simulink model "nmpc_controller"  (R2026a)
settings: Solver=FixedStepAuto  StopTime=Inf  FixedStep=0.05
PostLoadFcn:
  | if any(exist('dsrtsu_mdlpostloadfcn', 'file') ~= 0), dsrtsu_mdlpostloadfcn('Execute', bdroot); end
InitFcn:
  | , if any(exist('rtifpga_mdlclblib', 'file') ~= 0), rtifpga_mdlclblib('Init', bdroot); end,
  | , if any(exist('dsmpb_private', 'file') ~= 0), dsmpb_private('dsmpb_mdlclblib', 'Init', bdroot); end,
model workspace (MAT data in the model file):
  controllerConfig.schema_version = 1
  controllerConfig.vehicle.m = 1723
  controllerConfig.vehicle.Iz = 1960
  controllerConfig.vehicle.lf = 1.232
  controllerConfig.vehicle.lr = 1.468
  controllerConfig.vehicle.Cy = 62700
  controllerConfig.vehicle.track = 1.539
  controllerConfig.vehicle.Rw = 0.31
  controllerConfig.vehicle.g = 9.81
  controllerConfig.Ts = 0.05
  controllerConfig.N = 40
  controllerConfig.nx = 5
  controllerConfig.nu = 3
  controllerConfig.np = 19
  controllerConfig.W = [20  0  0  0  0  0  0  0; 0  50  0  0  0  0  0  0; 0  0  2  0  0  0  0  0; 0  0  0  0.1  0  0  0  0; 0  0  0  0  0.1  0  0  0; 0  0  0  0  0  1e-06  0  0; 0  0  0  0  0  0  1e-06  0; 0  0  0  0  0  0  0  1e-07]
  controllerConfig.We = [200  0  0  0  0; 0  500  0  0  0; 0  0  20  0  0; 0  0  0  1  0; 0  0  0  0  1]
  controllerConfig.lbu = [-9000; -9000; -6000]
  controllerConfig.ubu = [4500; 9000; 6000]
  controllerConfig.slack_linear = 1000
  controllerConfig.slack_quadratic = 1000
  controllerConfig.max_iter = 200
  controllerConfig.tolerance = 1e-06
  controllerConfig.qp_max_iter = 100
  controllerConfig.cond_N = 10
  initialUguess = [0  0  0  0  0  0  0  0  0  0  0  0  0  0  0  0  0  0  0  0  0  0  0  0  0  0  0  0  0  0  0  0  0  0  0  0  0  0  0  0; 0  0  0  0  0  0  0  0  0  0  0  0  0  0  0  0  0  0  0  0  0  0  0  0  0  0  0  0  0  0  0  0  0  0  0  0  0  0  0  0; 0  0  0  0  0  0  0  0  0  0  0  0  0  0  0  0  0  0  0  0  0  0  0  0  0  0  0  0  0  0  0  0  0  0  0  0  0  0  0  0]
  initialXguess = [-0.116260692271  -0.116260692271  -0.116260692271  -0.116260692271  -0.116260692271  -0.116260692271  -0.116260692271  -0.116260692271  -0.116260692271  -0.116260692271  -0.116260692271  -0.116260692271  -0.116260692271  -0.116260692271  -0.116260692271  -0.116260692271  -0.116260692271  -0.116260692271  -0.116260692271  -0.116260692271  -0.116260692271  -0.116260692271  -0.116260692271  -0.116260692271  -0.116260692271  -0.116260692271  -0.116260692271  -0.116260692271  -0.116260692271  -0.116260692271  -0.116260692271  -0.116260692271  -0.116260692271  -0.116260692271  -0.116260692271  -0.116260692271  -0.116260692271  -0.116260692271  -0.116260692271  -0.116260692271  -0.116260692271; -0.0164016572522  -0.0164016572522  -0.0164016572522  -0.0164016572522  -0.0164016572522  -0.0164016572522  -0.0164016572522  -0.0164016572522  -0.0164016572522  -0.0164016572522  -0.0164016572522  -0.0164016572522  -0.0164016572522  -0.0164016572522  -0.0164016572522  -0.0164016572522  -0.0164016572522  -0.0164016572522  -0.0164016572522  -0.0164016572522  -0.0164016572522  -0.0164016572522  -0.0164016572522  -0.0164016572522  -0.0164016572522  -0.0164016572522  -0.0164016572522  -0.0164016572522  -0.0164016572522  -0.0164016572522  -0.0164016572522  -0.0164016572522  -0.0164016572522  -0.0164016572522  -0.0164016572522  -0.0164016572522  -0.0164016572522  -0.0164016572522  -0.0164016572522  -0.0164016572522  -0.0164016572522; 0  0  0  0  0  0  0  0  0  0  0  0  0  0  0  0  0  0  0  0  0  0  0  0  0  0  0  0  0  0  0  0  0  0  0  0  0  0  0  0  0; 0  0  0  0  0  0  0  0  0  0  0  0  0  0  0  0  0  0  0  0  0  0  0  0  0  0  0  0  0  0  0  0  0  0  0  0  0  0  0  0  0; 0  0  0  0  0  0  0  0  0  0  0  0  0  0  0  0  0  0  0  0  0  0  0  0  0  0  0  0  0  0  0  0  0  0  0  0  0  0  0  0  0]
  instance.schema_version = 1
  instance.family_id = 1
  instance.instance_id = 1
  instance.seed = 1001
  instance.draws.uniform_draws = [0.306232179549 0.265063565608 0.196060063151 0.430521476567 0.0231135519921 0.195781915084 0.352805288469]
  instance.draws.e0_m = -0.116260692271
  instance.draws.psi0_rad = -0.0164016572522
  instance.draws.vx0_mps = 21.9606006315
  instance.draws.d0_m = 33.6104295313
  instance.draws.alead_mps2 = -5.93065934402
  instance.draws.vt_mps = 13.3310740371
  instance.draws.dt_m = 23.8201322117
  instance.draws.kc_per_m = 0
  instance.draws.curvature_choice_index = []
  instance.road.lane_width_m = 3.75
  instance.road.curvature_per_m = 0
  instance.road.bounds_m = [-1.75; 5.25]
  instance.friction_coefficient = 0.9
  instance.reference.speed_mps = 21.9606006315
  instance.timing.duration_s = 8
  instance.timing.controller_period_s = 0.05
  instance.timing.plant_step_s = 0.001
  instance.timing.number_of_control_samples = 160
  instance.ego.initial_state = [-0.116260692271; -0.0164016572522; 0; 0; 0]
  instance.ego.initial_longitudinal_speed_mps = 21.9606006315
  instance.ego.initial_station_m = 0
  instance.obstacles(1).initial_station_m = 33.6104295313
  instance.obstacles(1).lateral_position_m = 0
  instance.obstacles(1).initial_speed_mps = 21.9606006315
  instance.obstacles(1).acceleration_mps2 = -5.93065934402
  instance.obstacles(1).braking_start_s = 1
  instance.obstacles(2).initial_station_m = 23.8201322117
  instance.obstacles(2).lateral_position_m = 3.75
  instance.obstacles(2).initial_speed_mps = 13.3310740371
  instance.obstacles(2).acceleration_mps2 = 0
  instance.obstacles(2).braking_start_s = 0
  instance.obstacle_geometry.safety_semi_axes_m = [1.3; 4.5]
  instance.obstacle_geometry.collision_semi_axes_m = [0.9; 2.5]
  instance.termination.run_off_limit_m = 6
  laneData.schema_version = 1
  laneData.instance.schema_version = 1
  laneData.instance.family_id = 1
  laneData.instance.instance_id = 1
  laneData.instance.seed = 1001
  laneData.instance.draws.uniform_draws = [0.306232179549 0.265063565608 0.196060063151 0.430521476567 0.0231135519921 0.195781915084 0.352805288469]
  laneData.instance.draws.e0_m = -0.116260692271
  laneData.instance.draws.psi0_rad = -0.0164016572522
  laneData.instance.draws.vx0_mps = 21.9606006315
  laneData.instance.draws.d0_m = 33.6104295313
  laneData.instance.draws.alead_mps2 = -5.93065934402
  laneData.instance.draws.vt_mps = 13.3310740371
  laneData.instance.draws.dt_m = 23.8201322117
  laneData.instance.draws.kc_per_m = 0
  laneData.instance.draws.curvature_choice_index = []
  laneData.instance.road.lane_width_m = 3.75
  laneData.instance.road.curvature_per_m = 0
  laneData.instance.road.bounds_m = [-1.75; 5.25]
  laneData.instance.friction_coefficient = 0.9
  laneData.instance.reference.speed_mps = 21.9606006315
  laneData.instance.timing.duration_s = 8
  laneData.instance.timing.controller_period_s = 0.05
  laneData.instance.timing.plant_step_s = 0.001
  laneData.instance.timing.number_of_control_samples = 160
  laneData.instance.ego.initial_state = [-0.116260692271; -0.0164016572522; 0; 0; 0]
  laneData.instance.ego.initial_longitudinal_speed_mps = 21.9606006315
  laneData.instance.ego.initial_station_m = 0
  laneData.instance.obstacles(1).initial_station_m = 33.6104295313
  laneData.instance.obstacles(1).lateral_position_m = 0
  laneData.instance.obstacles(1).initial_speed_mps = 21.9606006315
  laneData.instance.obstacles(1).acceleration_mps2 = -5.93065934402
  laneData.instance.obstacles(1).braking_start_s = 1
  laneData.instance.obstacles(2).initial_station_m = 23.8201322117
  laneData.instance.obstacles(2).lateral_position_m = 3.75
  laneData.instance.obstacles(2).initial_speed_mps = 13.3310740371
  laneData.instance.obstacles(2).acceleration_mps2 = 0
  laneData.instance.obstacles(2).braking_start_s = 0
  laneData.instance.obstacle_geometry.safety_semi_axes_m = [1.3; 4.5]
  laneData.instance.obstacle_geometry.collision_semi_axes_m = [0.9; 2.5]
  laneData.instance.termination.run_off_limit_m = 6
  laneData.vehicle.m = 1723
  laneData.vehicle.Iz = 1960
  laneData.vehicle.lf = 1.232
  laneData.vehicle.lr = 1.468
  laneData.vehicle.Cy = 62700
  laneData.vehicle.track = 1.539
  laneData.vehicle.Rw = 0.31
  laneData.vehicle.g = 9.81
  laneData.lanes.schema_version = 1
  laneData.lanes.family_id = 1
  laneData.lanes.instance_id = 1
  laneData.lanes.station_m = [0 0.01 0.02 0.03 0.04 0.05 0.06 0.07 0.08 0.09 0.1 0.11 ... (50001 elements, 50001x1)]
  laneData.lanes.lane_width_m = 3.75
  laneData.lanes.number_of_lanes = 2
  laneData.lanes.curvature_per_m = 0
  laneData.lanes.origin_pose = [0; 0; 0]
  laneData.lanes.reference.X_m = [0 0.01 0.02 0.03 0.04 0.05 0.06 0.07 0.08 0.09 0.1 0.11 ... (50001 elements, 50001x1)]
  laneData.lanes.reference.Y_m = [0 0 0 0 0 0 0 0 0 0 0 0 ... (50001 elements, 50001x1)]
  laneData.lanes.reference.heading_rad = [0 0 0 0 0 0 0 0 0 0 0 0 ... (50001 elements, 50001x1)]
  laneData.lanes.boundaries.offsets_m = [-1.875; 1.875; 5.625]
  laneData.lanes.boundaries.X_m = [0 0.01 0.02 0.03 0.04 0.05 0.06 0.07 0.08 0.09 0.1 0.11 ... (150003 elements, 50001x3)]
  laneData.lanes.boundaries.Y_m = [-1.875 -1.875 -1.875 -1.875 -1.875 -1.875 -1.875 -1.875 -1.875 -1.875 -1.875 -1.875 ... (150003 elements, 50001x3)]
  laneData.lanes.centerlines.offsets_m = [0; 3.75]
  laneData.lanes.centerlines.X_m = [0 0.01 0.02 0.03 0.04 0.05 0.06 0.07 0.08 0.09 0.1 0.11 ... (100002 elements, 50001x2)]
  laneData.lanes.centerlines.Y_m = [0 0 0 0 0 0 0 0 0 0 0 0 ... (100002 elements, 50001x2)]
  laneData.lanes.controller_bounds.offsets_m = [-1.75; 5.25]
  laneData.lanes.controller_bounds.X_m = [0 0.01 0.02 0.03 0.04 0.05 0.06 0.07 0.08 0.09 0.1 0.11 ... (100002 elements, 50001x2)]
  laneData.lanes.controller_bounds.Y_m = [-1.75 -1.75 -1.75 -1.75 -1.75 -1.75 -1.75 -1.75 -1.75 -1.75 -1.75 -1.75 ... (100002 elements, 50001x2)]
  laneData.reference.station_m = [0 0.01 0.02 0.03 0.04 0.05 0.06 0.07 0.08 0.09 0.1 0.11 ... (50001 elements, 50001x1)]
  laneData.reference.X_m = [0 0.01 0.02 0.03 0.04 0.05 0.06 0.07 0.08 0.09 0.1 0.11 ... (50001 elements, 50001x1)]
  laneData.reference.Y_m = [0 0 0 0 0 0 0 0 0 0 0 0 ... (50001 elements, 50001x1)]
  laneData.reference.heading_rad = [0 0 0 0 0 0 0 0 0 0 0 0 ... (50001 elements, 50001x1)]
  laneData.reference.curvature_per_m = [0 0 0 0 0 0 0 0 0 0 0 0 ... (50001 elements, 50001x1)]
  laneData.reference.psi_pvr = [0 0 0 0 0 0 0 0 0 0 0 0 ... (50001 elements, 50001x1)]
  laneData.reference.dpsi_pr = [0 0 0 0 0 0 0 0 0 0 0 0 ... (50001 elements, 50001x1)]
  laneData.reference.dpsi_pvr = [0 0 0 0 0 0 0 0 0 0 0 0 ... (50001 elements, 50001x1)]
  laneData.reference.ddpsi_pr = [0 0 0 0 0 0 0 0 0 0 0 0 ... (50001 elements, 50001x1)]
  laneData.reference.ddpsi_pvr = [0 0 0 0 0 0 0 0 0 0 0 0 ... (50001 elements, 50001x1)]
  laneData.reference.vr = [21.9606006315 21.9606006315 21.9606006315 21.9606006315 21.9606006315 21.9606006315 21.9606006315 21.9606006315 21.9606006315 21.9606006315 21.9606006315 21.9606006315 ... (50001 elements, 50001x1)]
  laneData.reference.dvr = [0 0 0 0 0 0 0 0 0 0 0 0 ... (50001 elements, 50001x1)]
  laneData.reference.emin = [-1.75 -1.75 -1.75 -1.75 -1.75 -1.75 -1.75 -1.75 -1.75 -1.75 -1.75 -1.75 ... (50001 elements, 50001x1)]
  laneData.reference.emax = [5.25 5.25 5.25 5.25 5.25 5.25 5.25 5.25 5.25 5.25 5.25 5.25 ... (50001 elements, 50001x1)]
  mu = 0.9
PreSaveFcn:
  | , if any(exist('dsmpb_private', 'file') ~= 0), dsmpb_private('dsmpb_mdlclblib', 'PreSave', bdroot); end,
CloseFcn:
  | , if any(exist('dsmpb_private', 'file') ~= 0), dsmpb_private('dsmpb_mdlclblib', 'Close', bdroot); end,
settings Model: DataDictionary=vehicle_control.sldd  DSRTSU_INTERNAL_RTIFPGA=231  DSRTSU_INTERNAL_RTISTBM_VER=26.1  Creator=rayyu  LastModifiedBy=bxr240009
settings OptimizationCC: ConditionallyExecuteInputs=off  OptimizeBlockIOStorage=off  BufferReuse=off  InitFltsAndDblsToZero=on
settings DebuggingCC: TasksWithSamePriorityMsg=none
settings HardwareCC: ProdLargestAtomicInteger=Integer  ProdHWDeviceType=Custom Processor->Custom
settings ModelReferenceCC: EnableParallelModelReferenceBuilds=on
settings RTWCC: SystemTargetFile=dsrt.tlc  GenCodeOnly=on  TemplateMakefile=dsrt_default_tmf  RTWVerbose=off  Description=dSPACE Target DSRT - Generates SIC files for import by ConfigurationDesk and VEOS. Provides code generation for Simulink models imported in ConfigurationDesk.
settings RTWCC: CustomInclude=|
  | "C:\Users\bxr240009\Downloads\bim\real-time-performance-analysis\dependencies\acados-veos\include"
  | "C:\Users\bxr240009\Downloads\bim\real-time-performance-analysis\dependencies\acados-veos\include\blasfeo\include"
  | "C:\Users\bxr240009\Downloads\bim\real-time-performance-analysis\dependencies\acados-veos\include\hpipm\include"
settings RTWCC: CustomSource=|
  | C:\Users\bxr240009\Downloads\bim\real-time-performance-analysis\build\desktop\controller\c_generated_code\acados_sim_solver_ecu_vehicle_nmpc.c
  | C:\Users\bxr240009\Downloads\bim\real-time-performance-analysis\build\desktop\controller\c_generated_code\acados_solver_ecu_vehicle_nmpc.c
  | C:\Users\bxr240009\Downloads\bim\real-time-performance-analysis\build\desktop\controller\c_generated_code\ecu_vehicle_nmpc_constraints\ecu_vehicle_nmpc_constr_h_0_fun.c
  | C:\Users\bxr240009\Downloads\bim\real-time-performance-analysis\build\desktop\controller\c_generated_code\ecu_vehicle_nmpc_constraints\ecu_vehicle_nmpc_constr_h_0_fun_jac_uxt_zt.c
  | C:\Users\bxr240009\Downloads\bim\real-time-performance-analysis\build\desktop\controller\c_generated_code\ecu_vehicle_nmpc_constraints\ecu_vehicle_nmpc_constr_h_fun.c
  | C:\Users\bxr240009\Downloads\bim\real-time-performance-analysis\build\desktop\controller\c_generated_code\ecu_vehicle_nmpc_constraints\ecu_vehicle_nmpc_constr_h_fun_jac_uxt_zt.c
  | C:\Users\bxr240009\Downloads\bim\real-time-performance-analysis\build\desktop\controller\c_generated_code\ecu_vehicle_nmpc_cost\ecu_vehicle_nmpc_cost_y_0_fun.c
  | C:\Users\bxr240009\Downloads\bim\real-time-performance-analysis\build\desktop\controller\c_generated_code\ecu_vehicle_nmpc_cost\ecu_vehicle_nmpc_cost_y_0_fun_jac_ut_xt.c
  | C:\Users\bxr240009\Downloads\bim\real-time-performance-analysis\build\desktop\controller\c_generated_code\ecu_vehicle_nmpc_cost\ecu_vehicle_nmpc_cost_y_e_fun.c
  | C:\Users\bxr240009\Downloads\bim\real-time-performance-analysis\build\desktop\controller\c_generated_code\ecu_vehicle_nmpc_cost\ecu_vehicle_nmpc_cost_y_e_fun_jac_ut_xt.c
  | C:\Users\bxr240009\Downloads\bim\real-time-performance-analysis\build\desktop\controller\c_generated_code\ecu_vehicle_nmpc_cost\ecu_vehicle_nmpc_cost_y_fun.c
  | C:\Users\bxr240009\Downloads\bim\real-time-performance-analysis\build\desktop\controller\c_generated_code\ecu_vehicle_nmpc_cost\ecu_vehicle_nmpc_cost_y_fun_jac_ut_xt.c
  | C:\Users\bxr240009\Downloads\bim\real-time-performance-analysis\build\desktop\controller\c_generated_code\ecu_vehicle_nmpc_model\ecu_vehicle_nmpc_expl_ode_fun.c
  | C:\Users\bxr240009\Downloads\bim\real-time-performance-analysis\build\desktop\controller\c_generated_code\ecu_vehicle_nmpc_model\ecu_vehicle_nmpc_expl_vde_adj.c
  | C:\Users\bxr240009\Downloads\bim\real-time-performance-analysis\build\desktop\controller\c_generated_code\ecu_vehicle_nmpc_model\ecu_vehicle_nmpc_expl_vde_forw.c
settings RTWCC: CustomLibrary=|
  | "C:\Users\bxr240009\Downloads\bim\real-time-performance-analysis\dependencies\acados-veos\lib\acados.lib"
  | "C:\Users\bxr240009\Downloads\bim\real-time-performance-analysis\dependencies\acados-veos\lib\blasfeo.lib"
  | "C:\Users\bxr240009\Downloads\bim\real-time-performance-analysis\dependencies\acados-veos\lib\hpipm.lib"
settings STFCustomTargetCC: SystemTargetFile=dsrt.tlc  MultiwordLength=2048.0  ParMdlRefBuildCompliant=on  GRTInterface=off  DSTargetArchitecture=32-bit  TRCGenerateVirtualBlocks=off  TRCGenerateLabels=off  TRCOnlyGlobals=off  VDFType=TRC  TRCGenerateParamValues=off  TRCGenerateDerivatives=off  TRCGenerateStates=off  TRCIsOmitVdOn=on
settings GRTTargetCC: CompOptLevelCompliant=off  ConcurrentExecutionCompliant=off  CombineOutputUpdateFcns=off  MatFileLogging=off  CPPClassGenCompliant=off

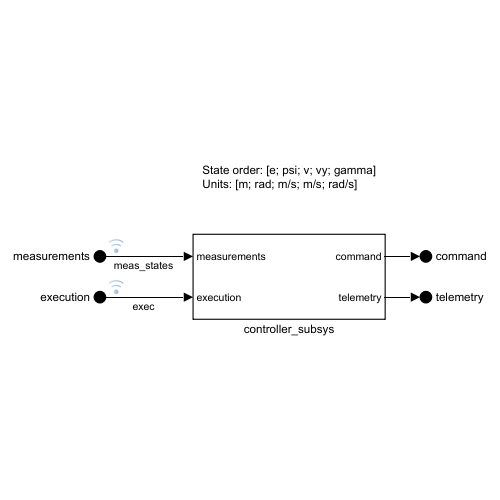
[thumbnail: Simulink's stored preview of the top-level diagram]
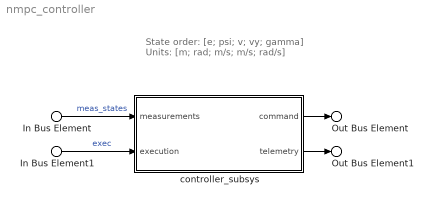
== system nmpc_controller ==
  note: State order: [e; psi; v; vy; gamma]
      | Units: [m; rad; m/s; m/s; rad/s]
  In Bus Element : Inport  PortName=measurements
  In Bus Element1 : Inport  Port=2  PortName=execution
  controller_subsys : Subsystem
  Out Bus Element : Outport  PortName=command
  Out Bus Element1 : Outport  Port=2  PortName=telemetry
  wires:
  In Bus Element/1 -> controller_subsys/1(measurements)  "meas_states"
  In Bus Element1/1 -> controller_subsys/2(execution)  "exec"
  controller_subsys/1(command) -> Out Bus Element/1
  controller_subsys/2(telemetry) -> Out Bus Element1/1

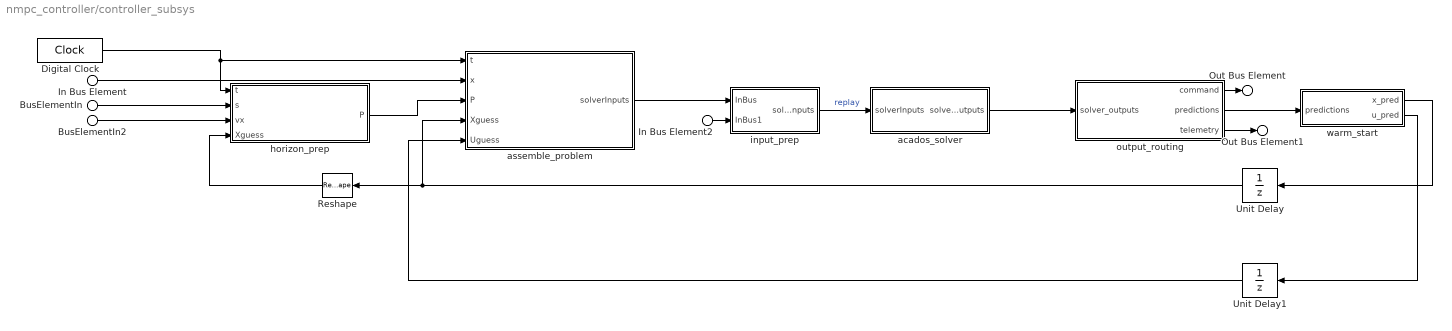
== system nmpc_controller/controller_subsys ==
  In Bus Element : Inport  PortName=measurements  Element=x
  BusElementIn2 : Inport  PortName=measurements  Element=vx
  BusElementIn : Inport  PortName=measurements  Element=s
  In Bus Element2 : Inport  Port=2  PortName=execution
  Digital Clock : DigitalClock  SampleTime=0.05
  Reshape : Reshape  OutputDimensionality=Customize  OutputDimensions=[205,1]
  Unit Delay : UnitDelay  SampleTime=0.05
  Unit Delay1 : UnitDelay  SampleTime=0.05
  acados_solver : Subsystem
  assemble_problem : MATLAB Function  TreatAsAtomicUnit=on
  horizon_prep : MATLAB Function  TreatAsAtomicUnit=on
  input_prep : Subsystem
  output_routing : Subsystem
  warm_start : Subsystem
  Out Bus Element : Outport  PortName=command
  Out Bus Element1 : Outport  Port=2  PortName=telemetry
  wires:
  acados_solver/1(solver_outputs) -> output_routing/1(solver_outputs)
  In Bus Element/1 -> assemble_problem/2(x)
  assemble_problem/1(solverInputs) -> input_prep/1(InBus)
  output_routing/2(predictions) -> warm_start/1(predictions)
  warm_start/1(x_pred) -> Unit Delay/1
  warm_start/2(u_pred) -> Unit Delay1/1
  input_prep/1(solverInputs) -> acados_solver/1(solverInputs)  "replay"
  horizon_prep/1(P) -> assemble_problem/3(P)
  BusElementIn2/1 -> horizon_prep/3(vx)
  BusElementIn/1 -> horizon_prep/2(s)
  output_routing/1(command) -> Out Bus Element/1
  output_routing/3(telemetry) -> Out Bus Element1/1
  In Bus Element2/1 -> input_prep/2(InBus1)
  Digital Clock/1 -> horizon_prep/1(t), assemble_problem/1(t)
  Unit Delay/1 -> assemble_problem/4(Xguess), Reshape/1
  Unit Delay1/1 -> assemble_problem/5(Uguess)
  Reshape/1 -> horizon_prep/4(Xguess)

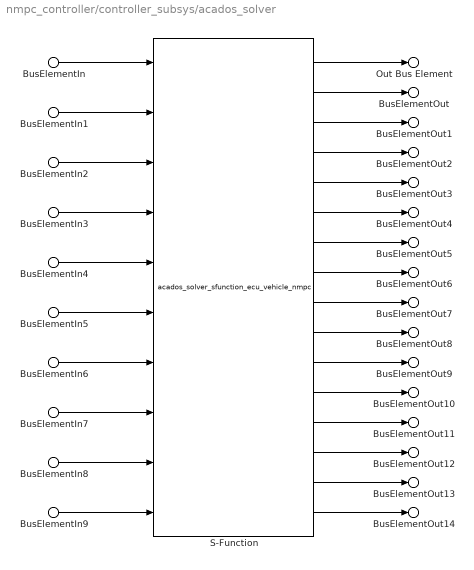
== system nmpc_controller/controller_subsys/acados_solver ==
  BusElementIn : Inport  PortName=solverInputs  Element=lbx_0
  BusElementIn1 : Inport  PortName=solverInputs  Element=ubx_0
  BusElementIn2 : Inport  PortName=solverInputs  Element=parameter_traj
  BusElementIn3 : Inport  PortName=solverInputs  Element=lh
  BusElementIn4 : Inport  PortName=solverInputs  Element=uh
  BusElementIn5 : Inport  PortName=solverInputs  Element=lh_0
  BusElementIn6 : Inport  PortName=solverInputs  Element=uh_0
  BusElementIn7 : Inport  PortName=solverInputs  Element=x_init
  BusElementIn8 : Inport  PortName=solverInputs  Element=u_init
  BusElementIn9 : Inport  PortName=solverInputs  Element=iter_cap
  S-Function : S-Function  FunctionName=acados_solver_sfunction_ecu_vehicle_nmpc  SFunctionDeploymentMode=off  EnableBusSupport=off
  Out Bus Element : Outport  PortName=solver_outputs  Element=u0
  BusElementOut : Outport  PortName=solver_outputs  Element=utraj
  BusElementOut1 : Outport  PortName=solver_outputs  Element=xtraj
  BusElementOut2 : Outport  PortName=solver_outputs  Element=slack_values
  BusElementOut3 : Outport  PortName=solver_outputs  Element=solver_status
  BusElementOut4 : Outport  PortName=solver_outputs  Element=cost_value
  BusElementOut5 : Outport  PortName=solver_outputs  Element=kkt_residuals
  BusElementOut6 : Outport  PortName=solver_outputs  Element=x1
  BusElementOut7 : Outport  PortName=solver_outputs  Element=cpu_time
  BusElementOut8 : Outport  PortName=solver_outputs  Element=cpu_time_qp
  BusElementOut9 : Outport  PortName=solver_outputs  Element=cpu_time_lin
  BusElementOut10 : Outport  PortName=solver_outputs  Element=sqp_iter
  BusElementOut11 : Outport  PortName=solver_outputs  Element=qp_iteration_history
  BusElementOut12 : Outport  PortName=solver_outputs  Element=residual_history
  BusElementOut13 : Outport  PortName=solver_outputs  Element=history_length
  BusElementOut14 : Outport  PortName=solver_outputs  Element=lam_stage0
  wires:
  BusElementIn4/1 -> S-Function/5
  BusElementIn2/1 -> S-Function/3
  BusElementIn8/1 -> S-Function/9
  BusElementIn6/1 -> S-Function/7
  BusElementIn5/1 -> S-Function/6
  BusElementIn7/1 -> S-Function/8
  BusElementIn1/1 -> S-Function/2
  BusElementIn/1 -> S-Function/1
  BusElementIn3/1 -> S-Function/4
  BusElementIn9/1 -> S-Function/10
  S-Function/9 -> BusElementOut7/1
  S-Function/1 -> Out Bus Element/1
  S-Function/15 -> BusElementOut13/1
  S-Function/14 -> BusElementOut12/1
  S-Function/3 -> BusElementOut1/1
  S-Function/4 -> BusElementOut2/1
  S-Function/8 -> BusElementOut6/1
  S-Function/2 -> BusElementOut/1
  S-Function/7 -> BusElementOut5/1
  S-Function/16 -> BusElementOut14/1
  S-Function/10 -> BusElementOut8/1
  S-Function/13 -> BusElementOut11/1
  S-Function/6 -> BusElementOut4/1
  S-Function/12 -> BusElementOut10/1
  S-Function/11 -> BusElementOut9/1
  S-Function/5 -> BusElementOut3/1

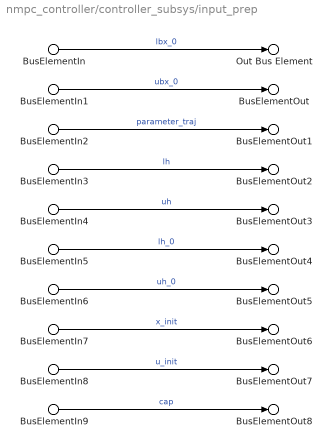
== system nmpc_controller/controller_subsys/input_prep ==
  BusElementIn : Inport  PortName=InBus  Element=lbx_0
  BusElementIn1 : Inport  PortName=InBus  Element=ubx_0
  BusElementIn2 : Inport  PortName=InBus  Element=parameter_traj
  BusElementIn3 : Inport  PortName=InBus  Element=lh
  BusElementIn4 : Inport  PortName=InBus  Element=uh
  BusElementIn5 : Inport  PortName=InBus  Element=lh_0
  BusElementIn6 : Inport  PortName=InBus  Element=uh_0
  BusElementIn7 : Inport  PortName=InBus  Element=x_init
  BusElementIn8 : Inport  PortName=InBus  Element=u_init
  BusElementIn9 : Inport  Port=2  PortName=InBus1  Element=cap
  Out Bus Element : Outport  PortName=solverInputs  Element=lbx_0
  BusElementOut : Outport  PortName=solverInputs  Element=ubx_0
  BusElementOut1 : Outport  PortName=solverInputs  Element=parameter_traj
  BusElementOut2 : Outport  PortName=solverInputs  Element=lh
  BusElementOut3 : Outport  PortName=solverInputs  Element=uh
  BusElementOut4 : Outport  PortName=solverInputs  Element=lh_0
  BusElementOut5 : Outport  PortName=solverInputs  Element=uh_0
  BusElementOut6 : Outport  PortName=solverInputs  Element=x_init
  BusElementOut7 : Outport  PortName=solverInputs  Element=u_init
  BusElementOut8 : Outport  PortName=solverInputs  Element=iter_cap
  wires:
  BusElementIn/1 -> Out Bus Element/1  "lbx_0"
  BusElementIn1/1 -> BusElementOut/1  "ubx_0"
  BusElementIn2/1 -> BusElementOut1/1  "parameter_traj"
  BusElementIn3/1 -> BusElementOut2/1  "lh"
  BusElementIn4/1 -> BusElementOut3/1  "uh"
  BusElementIn5/1 -> BusElementOut4/1  "lh_0"
  BusElementIn6/1 -> BusElementOut5/1  "uh_0"
  BusElementIn7/1 -> BusElementOut6/1  "x_init"
  BusElementIn8/1 -> BusElementOut7/1  "u_init"
  BusElementIn9/1 -> BusElementOut8/1  "cap"

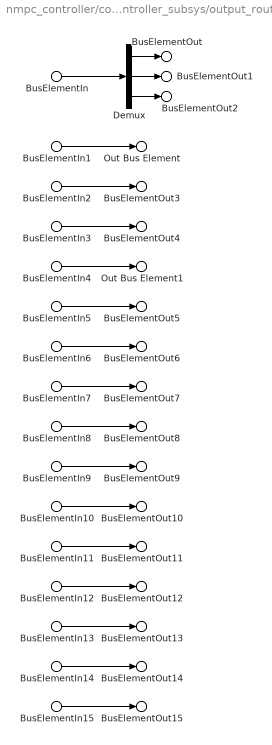
== system nmpc_controller/controller_subsys/output_routing ==
  BusElementIn : Inport  PortName=solver_outputs  Element=u0
  BusElementIn1 : Inport  PortName=solver_outputs  Element=utraj
  BusElementIn2 : Inport  PortName=solver_outputs  Element=xtraj
  BusElementIn4 : Inport  PortName=solver_outputs  Element=slack_values
  BusElementIn5 : Inport  PortName=solver_outputs  Element=solver_status
  BusElementIn6 : Inport  PortName=solver_outputs  Element=cost_value
  BusElementIn7 : Inport  PortName=solver_outputs  Element=kkt_residuals
  BusElementIn3 : Inport  PortName=solver_outputs  Element=x1
  BusElementIn8 : Inport  PortName=solver_outputs  Element=cpu_time
  BusElementIn9 : Inport  PortName=solver_outputs  Element=cpu_time_qp
  BusElementIn10 : Inport  PortName=solver_outputs  Element=cpu_time_lin
  BusElementIn11 : Inport  PortName=solver_outputs  Element=sqp_iter
  BusElementIn12 : Inport  PortName=solver_outputs  Element=qp_iteration_history
  BusElementIn13 : Inport  PortName=solver_outputs  Element=residual_history
  BusElementIn14 : Inport  PortName=solver_outputs  Element=history_length
  BusElementIn15 : Inport  PortName=solver_outputs  Element=lam_stage0
  Demux : Demux  Outputs=3
  BusElementOut : Outport  PortName=command  Element=Fx
  BusElementOut1 : Outport  PortName=command  Element=Fy
  BusElementOut2 : Outport  PortName=command  Element=Mz
  Out Bus Element : Outport  Port=2  PortName=predictions  Element=utraj
  BusElementOut3 : Outport  Port=2  PortName=predictions  Element=xtraj
  BusElementOut4 : Outport  Port=2  PortName=predictions  Element=x1
  Out Bus Element1 : Outport  Port=3  PortName=telemetry  Element=slack_values
  BusElementOut5 : Outport  Port=3  PortName=telemetry  Element=solver_status
  BusElementOut6 : Outport  Port=3  PortName=telemetry  Element=cost_value
  BusElementOut7 : Outport  Port=3  PortName=telemetry  Element=kkt_residuals
  BusElementOut8 : Outport  Port=3  PortName=telemetry  Element=cpu_time
  BusElementOut9 : Outport  Port=3  PortName=telemetry  Element=cpu_time_qp
  BusElementOut10 : Outport  Port=3  PortName=telemetry  Element=cpu_time_lin
  BusElementOut11 : Outport  Port=3  PortName=telemetry  Element=sqp_iter
  BusElementOut12 : Outport  Port=3  PortName=telemetry  Element=qp_iteration_history
  BusElementOut13 : Outport  Port=3  PortName=telemetry  Element=residual_history
  BusElementOut14 : Outport  Port=3  PortName=telemetry  Element=history_length
  BusElementOut15 : Outport  Port=3  PortName=telemetry  Element=lam_stage0
  wires:
  BusElementIn/1 -> Demux/1
  Demux/1 -> BusElementOut/1
  Demux/2 -> BusElementOut1/1
  Demux/3 -> BusElementOut2/1
  BusElementIn1/1 -> Out Bus Element/1
  BusElementIn2/1 -> BusElementOut3/1
  BusElementIn3/1 -> BusElementOut4/1
  BusElementIn5/1 -> BusElementOut5/1
  BusElementIn6/1 -> BusElementOut6/1
  BusElementIn7/1 -> BusElementOut7/1
  BusElementIn8/1 -> BusElementOut8/1
  BusElementIn9/1 -> BusElementOut9/1
  BusElementIn10/1 -> BusElementOut10/1
  BusElementIn11/1 -> BusElementOut11/1
  BusElementIn4/1 -> Out Bus Element1/1
  BusElementIn12/1 -> BusElementOut12/1
  BusElementIn13/1 -> BusElementOut13/1
  BusElementIn14/1 -> BusElementOut14/1
  BusElementIn15/1 -> BusElementOut15/1

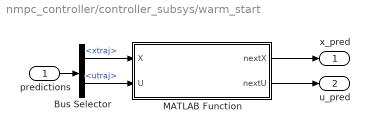
== system nmpc_controller/controller_subsys/warm_start ==
  predictions : Inport
  Bus Selector : BusSelector  OutputSignals=xtraj,utraj
  MATLAB Function : MATLAB Function  TreatAsAtomicUnit=on
  x_pred : Outport
  u_pred : Outport  Port=2
  wires:
  predictions/1 -> Bus Selector/1
  MATLAB Function/1(nextX) -> x_pred/1
  Bus Selector/1 -> MATLAB Function/1(X)  "<xtraj>"
  Bus Selector/2 -> MATLAB Function/2(U)  "<utraj>"
  MATLAB Function/2(nextU) -> u_pred/1

== matlab function nmpc_controller/controller_subsys/warm_start/MATLAB Function ==
  data: X input; nextX output; U input; nextU output
function [nextX, nextU] = shiftWarmStart(X, U)
% Shift the previous solution using the shared MATLAB implementation.

warmStart = ecu.control.shift_warm_start(X, U);

nextX = warmStart.x;
nextU = warmStart.u;

end

== matlab function nmpc_controller/controller_subsys/assemble_problem ==
  data: t input; x input size=[5 1]; solverInputs output Bus: SolverInputBus; P input size=[19 41]; Xguess input size=[5 41]; Uguess input size=[3 40]; controllerConfig parameter; mu parameter
function solverInputs = assembleProblem( ...
    t, x, P, Xguess, Uguess, controllerConfig, mu)

warmStart.x = Xguess;
warmStart.u = Uguess;

ports = ecu.control.format_simulink_inputs( ...
    x, P, mu, warmStart, controllerConfig);

% Arrange fields in the solver adapter's input order.
solverInputs.lbx_0 = ports.lbx_0;
solverInputs.ubx_0 = ports.ubx_0;
solverInputs.parameter_traj = ports.parameter_traj;

solverInputs.lh = ports.lh;
solverInputs.uh = ports.uh;
solverInputs.lh_0 = ports.lh_0;
solverInputs.uh_0 = ports.uh_0;

solverInputs.x_init = ports.x_init;
solverInputs.u_init = ports.u_init;
solverInputs.iter_cap = double(controllerConfig.max_iter);

end

== matlab function nmpc_controller/controller_subsys/horizon_prep ==
  data: t input double size=1; P output; s input size=1; vx input size=1; Xguess input size=[205 1]; controllerConfig parameter; instance parameter
function P = buildHorizon( ...
    t, s, vx, Xguess, controllerConfig, instance)
% Build the stage parameters for the current controller execution.
assert(numel(Xguess) == 205);
Xmatrix = reshape(Xguess, 5, 41);
previousSpeedErrors = Xmatrix(3, 1:40);
% Use the existing A6 analytical reference and obstacle prediction.
P = ecu.scenario.prepare_horizon( ...
    instance, ...
    t, ...
    s, ...
    vx, ...
    previousSpeedErrors, ...
    controllerConfig);

end
